simulink model "Maxom_fcs_noncascaded"  (R2025b)
settings: Solver=ode45  StartTime=0.0  StopTime=0.30  FixedStep=1e-6  MaxStep=1e-5  RelTol=1e-4  EnableMultiTasking=on
values from neighbouring files (symbols this model uses):
  Bfric = 0    [PMSMpara.m]
  ffai = 0.008667    [PMSMpara.m]
  Imax = 20    [PMSMpara.m]
  J = 0.044e-4    (= 4.4e-06)    [PMSMpara.m]
  kis = 0    [PMSMpara.m]
  kps = fsc*6.28*J/Kt    (= 0.364364007978)    [PMSMpara.m]
  Kt = np*1.5*ffai    (= 0.0910035)    [PMSMpara.m]
  Ld = Ls    (= 0.00045)    [PMSMpara.m]
  Lq = Ls    (= 0.00045)    [PMSMpara.m]
  np = 7    [PMSMpara.m]
  Rs = 0.5    [PMSMpara.m]
  Tcur = 1/32000    (= 3.125e-05)    [PMSMpara.m]
  Tpwm = 1/32000    (= 3.125e-05)    [PMSMpara.m]
  Tspd = 1/32000    (= 3.125e-05)    [PMSMpara.m]
  wn = 311040    [PMSMpara.m]
  zeta = 1    [PMSMpara.m]
undefined symbols (not defined in the file or in its folder): dspblkCoreblockFVToolHelper, gcbh
libraries: simulink x4, slpidlib x2, spsUniversalBridgeLib x1, spsCurrentMeasurementLib x1, EasyGo_Machine_lib x1, spsPermanentMagnetSynchronousMachineLib x1, spsSVPWMGenerator2LevelLib x1, spsDCVoltageSourceLib x1, sps_lib x1
(part 2 of 4)

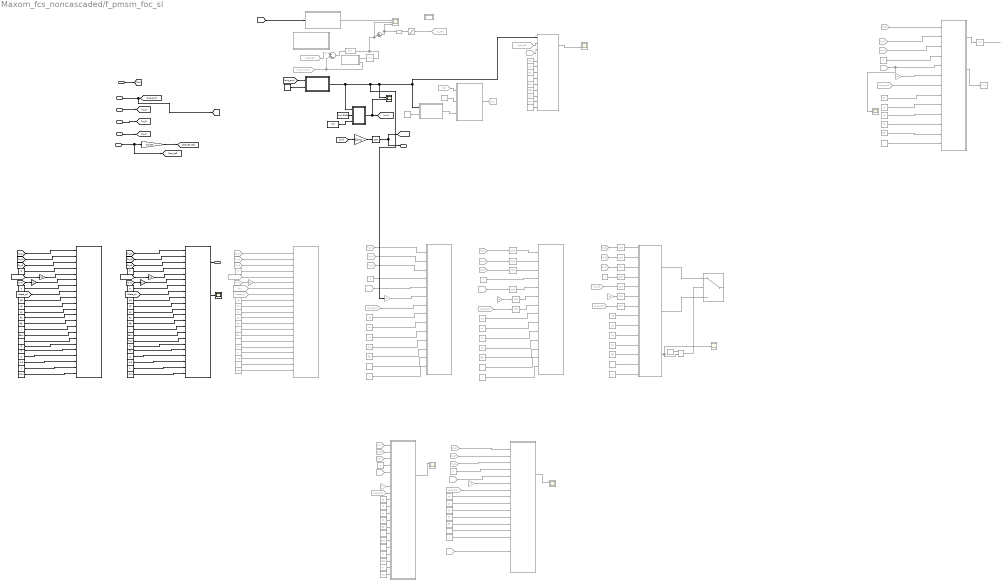
== system Maxom_fcs_noncascaded/f_pmsm_foc_sl ==
  note: This is non-cascaded, clearer to read but takes aroun 200e-6s to compute.
  note: ripple pzdc
      | but needs 20e-6 to calculate ggs
  note: 速度环控制器+电流前馈
  note: computational time around 200ms. good performance, however still the ripple ~20% exists
  note: performance same as smdo+1step, but has apendix
  note: same as the one on the right but loops were optimized and the matrix multiplication was taken out 70e-6s to compute, a little worse performn.
  Is_A : Inport  SampleTime=Tpwm
  Is_B : Inport  Port=2  SampleTime=Tpwm
  Is_C : Inport  Port=3  SampleTime=Tpwm
  ang_enc : Inport  Port=4  OutDataTypeStr=single  SampleTime=Tpwm
  spd_ref : Inport  Port=5  SampleTime=Tpwm
  Te : Inport  Port=6  SampleTime=Tpwm
  " lpf_2nd3" : Subsystem  mask{ts=Tpwm}
      mask prompts: ts "Sample time"
      mask DialogControl DescGroupVar Prompt: 2nd order low-pass filter
  Constant{,55,69,74} (4 alike) : Constant  Commented=on  Value=J
  Constant{1,5,21,24,33,45,62} (7 alike) : Constant  Commented=on  Value=Ld
  Constant{2,10,19,22,25,34,66} (7 alike) : Constant  Commented=on  Value=Lq
  Constant100 : Constant  Value=ffai
  Constant101 : Constant  Value=48
  Constant{86,90,94,102,106,110} (6 alike) : Constant  Value=0
  Constant103 : Constant  Value=Bfric
  Constant104 : Constant  Value=J
  Constant105 : Constant  Value=5
  Constant107 : Constant  Value=0.8
  Constant108 : Constant
  Constant109 : Constant  Value=Imax
  Constant{3,11,20,26,35,46,67} (7 alike) : Constant  Commented=on  Value=Rs
  Constant111 : Constant  Value=3
  Constant{4,12,27,36,40,48,58,68} (8 alike) : Constant  Commented=on  Value=Tpwm
  Constant{13,37,41,49,78} (5 alike) : Constant  Commented=on
  Constant{6,14,29,38,42,50,60,70} (8 alike) : Constant  Commented=on  Value=ffai
  Constant{7,15,30,39,43,51,71} (7 alike) : Constant  Commented=on  Value=48
  Constant{8..9,16,23,32,44,72,76} (8 alike) : Constant  Commented=on  Value=0
  Constant17 : Constant  Value=2*pi*6000  OutDataTypeStr=single
  Constant18 : Constant  Value=0.8  OutDataTypeStr=single
  Constant28 : Constant  Commented=on  Value=2
  Constant31 : Constant  Value=Tpwm  OutDataTypeStr=single
  Constant47 : Constant  Commented=on  Value=Bfric
  Constant52 : Constant  Commented=on  Value=zeta
  Constant53 : Constant  Commented=on  Value=wn
  Constant54 : Constant  Commented=on  Value=Imax
  Constant56 : Constant  Commented=on  Value=Tpwm  OutDataTypeStr=single
  Constant57 : Constant  Commented=on  Value=kis
  Constant59 : Constant  Commented=on  Value=Imax
  Constant61 : Constant  Commented=on  Value=kps
  Constant63 : Constant  Commented=on  Value=Bfric
  Constant64 : Constant  Commented=on  Value=zeta
  Constant65 : Constant  Commented=on  Value=wn
  Constant73 : Constant  Commented=on  Value=Bfric
  Constant75 : Constant  Commented=on  Value=5
  Constant77 : Constant  Commented=on  Value=0.8
  Constant79 : Constant  Commented=on  Value=Imax
  Constant80 : Constant  Value=Ld
  Constant81 : Constant  Value=Lq
  Constant82 : Constant  Value=Rs
  Constant83 : Constant  Value=Tcur
  Constant84 : Constant  Value=ffai
  Constant85 : Constant  Value=48
  Constant87 : Constant  Value=Bfric
  Constant88 : Constant  Value=J
  Constant89 : Constant  Value=5
  Constant91 : Constant  Value=0.8
  Constant92 : Constant
  Constant93 : Constant  Value=Imax
  Constant95 : Constant  Value=3
  Constant96 : Constant  Value=Ld
  Constant97 : Constant  Value=Lq
  Constant98 : Constant  Value=Rs
  Constant99 : Constant  Value=Tpwm
  Data Type Conversion : DataTypeConversion  Commented=on  SaturateOnIntegerOverflow=off  RndMeth=Floor
  Delay1 : Delay  Commented=on  DelayLength=1  InitialCondition=0  SampleTime=Tpwm
  Delay2 : Delay  Commented=on  DelayLength=1  InitialCondition=0  SampleTime=Tcur
  Delay3 : Delay  Commented=on  DelayLength=1  InitialCondition=0  SampleTime=Tcur
  Filter_13k : Subsystem  Tag=FilterWizardSubSystem  Commented=on
      settings: ErrorFcn=dspFilterRealizedInBasicElemsAlgLoopErrFcnCallback
  From{,13..14,26} (4 alike) : From  Commented=on  GotoTag=spd_ref
  From{1,6,17,21,24,31,37} (7 alike) : From  Commented=on  GotoTag=is_c
  From10 : From  Commented=on  GotoTag=wm_syn_rpm  TagVisibility=global
  From{5,12,36,42..43} (5 alike) : From  Commented=on  GotoTag=iq_ref
  From15 : From  Commented=on  GotoTag=wm
  From{2,7,18,22,28,32,38} (7 alike) : From  Commented=on  GotoTag=is_a
  From{3,8,19,23,29,33,39} (7 alike) : From  Commented=on  GotoTag=is_b
  From{4,9,20,25,35,41} (6 alike) : From  Commented=on  GotoTag=ang_enc
  From27 : From  Commented=on  GotoTag=T_load
  From30 : From  Commented=on  GotoTag=theta_e
  From34 : From  Commented=on  GotoTag=spd_ref_rad
  From40 : From  Commented=on  GotoTag=TL
  From44 : From  Commented=on  GotoTag=Te
  Gain{1..4,7,10,16} (7 alike) : Gain  Commented=on  Gain=np
  Gain14 : Gain  Gain=60/np
  Gain26 : Gain  Gain=2*pi/60
  Gain5 : Gain  Gain=np*0.895
  Gain6 : Gain  Gain=np
  Gain8 : Gain  Gain=np*0.9
  Gain9 : Gain  Gain=np
  Goto10 : Goto  Commented=on  GotoTag=iq_ref
  Goto2 : Goto  Commented=on  GotoTag=TL
  MATLAB Function : MATLAB Function  Commented=on  TreatAsAtomicUnit=on
  MATLAB Function1 : MATLAB Function  Commented=on  TreatAsAtomicUnit=on
  MATLAB Function10 : MATLAB Function  Commented=on  TreatAsAtomicUnit=on  SystemSampleTime=1/16000
  MATLAB Function11 : MATLAB Function  Commented=on  TreatAsAtomicUnit=on
  MATLAB Function12 : MATLAB Function  TreatAsAtomicUnit=on  SystemSampleTime=Tpwm
  MATLAB Function13 : MATLAB Function  TreatAsAtomicUnit=on  SystemSampleTime=Tpwm
  MATLAB Function2 : MATLAB Function  Commented=on  TreatAsAtomicUnit=on
  MATLAB Function3 : MATLAB Function  Commented=on  TreatAsAtomicUnit=on
  MATLAB Function4 : MATLAB Function  Commented=on  TreatAsAtomicUnit=on  SystemSampleTime=1/16000
  MATLAB Function5 : MATLAB Function  Commented=on  TreatAsAtomicUnit=on  SystemSampleTime=1/16000
  MATLAB Function6 : MATLAB Function  TreatAsAtomicUnit=on
  MATLAB Function7 : MATLAB Function  Commented=on  TreatAsAtomicUnit=on
  MATLAB Function8 : MATLAB Function  Commented=on  TreatAsAtomicUnit=on  SystemSampleTime=1/16000
  MATLAB Function9 : MATLAB Function  Commented=on  TreatAsAtomicUnit=on
  PID Controller : slpidlib/PID Controller  Commented=on  Controller=PI  Form=Parallel  TimeDomain=Discrete-time  UseExternalTs=off  SampleTime=Tpwm  IntegratorMethod=Forward Euler  FilterMethod=Forward Euler  ControllerParametersSource=internal  P=0.044e-4*2*pi*2500  I=0.0001*4.5*0.2*2*10  UseKiTs=off  D=0  UseExternalDerivativeSource=off  N=100  UseFilter=on  TunerSelectOption=Transfer Function Based (PID Tuner App)  InitialConditionSource=internal  InitialConditionForIntegrator=0  InitialConditionForFilter=0  DifferentiatorICPrevScaledInput=0  ExternalReset=none  TrackingMode=off  Kt=1  LimitOutput=on  SatLimitsSource=internal  UpperSaturationLimit=20  LowerSaturationLimit=-20  LinearizeAsGain=on  AntiWindupMode=clamping  Kb=0.1  LimitIntegrator=off  UpperIntegratorSaturationLimit=20  LowerIntegratorSaturationLimit=-20  POutMin=[]  POutMax=[]  IOutMin=[]  IOutMax=[]  DOutMin=[]  DOutMax=[]  NOutMin=[]  NOutMax=[]  SumOutMin=[]  SumOutMax=[]  SaturationOutMin=[]  SaturationOutMax=[]  PParamMin=[]  PParamMax=[]  IParamMin=[]  IParamMax=[]  DParamMin=[]  DParamMax=[]  NParamMin=[]  NParamMax=[]  KbParamMin=[]  KbParamMax=[]  KtParamMin=[]  KtParamMax=[]  KbOutMin=[]  KbOutMax=[]  KtOutMin=[]  KtOutMax=[]  IntegratorOutMin=[]  IntegratorOutMax=[]  FilterOutMin=[]  FilterOutMax=[]  SumI1OutMin=[]  SumI1OutMax=[]  SumI2OutMin=[]  SumI2OutMax=[]  SumI3OutMin=[]  SumI3OutMax=[]  SumI4OutMin=[]  SumI4OutMax=[]  SumDOutMin=[]  SumDOutMax=[]  DifferentiatorOutMin=[]  DifferentiatorOutMax=[]  FilterDiffOutCoefMin=[]  FilterDiffOutCoefMax=[]  ReciprocalOutMin=[]  ReciprocalOutMax=[]  SumDenOutMin=[]  SumDenOutMax=[]  SumNumOutMin=[]  SumNumOutMax=[]  DivideOutMin=[]  DivideOutMax=[]  UdiffTsProdOutMin=[]  UdiffTsProdOutMax=[]  NTsProdOutMin=[]  NTsProdOutMax=[]  UintegralTsProdOutMin=[]  UintegralTsProdOutMax=[]  UngainTsProdOutMin=[]  UngainTsProdOutMax=[]  ClampingZeroOutDataTypeStr=Inherit: Inherit via back propagation  ClampingZeroOutMin=[]  ClampingZeroOutMax=[]  FilterDenConstantOutDataTypeStr=Inherit: Inherit via back propagation  FilterDenConstantOutMin=[]  FilterDenConstantOutMax=[]  PCopyOutDataTypeStr=Inherit: Inherit via back propagation  PCopyOutMin=[]  PCopyOutMax=[]  NCopyOutDataTypeStr=Inherit: Inherit via back propagation  NCopyOutMin=[]  NCopyOutMax=[]  IntegratorContinuousStateAttributes=''  IntegratorStateMustResolveToSignalObject=off  IntegratorRTWStateStorageClass=Auto  FilterContinuousStateAttributes=''  FilterStateMustResolveToSignalObject=off  FilterRTWStateStorageClass=Auto  ParallelPVariant=InternalParameters  IdealPVariant=Disabled  IVariant=InternalParameters  DVariant=Disabled  IntegratorVariant=Discrete  SatVariant=Enabled  AWVariant=DiscClampingParallel  PCopyVariant=Disabled  TRVariant=Disabled  FdbkBlocksVariant=Forward  IdealPFdbkVariant=Disabled  SatFdbkVariant=Disabled  DerivativeFilterVariant=Disabled  NVariant=Disabled  NCopyVariant=Disabled_SignalSpec  FilterICVariant=Disabled  IntegratorICVariant=InternalICs  ExternalResetVariant=Disabled  TRSumVariant=Passthrough  SumFdbkVariant=Disabled  SumVariant=Sum_PI  TsampFilterVariant=InternalTs  TsampNgainVariant=Passthrough  TsampIntegralVariant=Disabled_SignalSpec  ExternalSaturationOutDataTypeStr=Inherit: Same as second input  DerivativeSourceVariant=Disabled  PreIntVariant=InternalPreInt
  Relational Operator : RelationalOperator  Commented=on  Operator=<  OutDataTypeStr=boolean  RndMeth=Simplest  InputSameDT=off
  Repeating Sequence2 : simulink/Sources/Repeating Sequence  Commented=on  rep_seq_t=[0 Tpwm]  rep_seq_y=[0 1]
  Saturation : Saturate  Commented=on  UpperLimit=20  LowerLimit=-20
  Scope : Scope  Commented=on  NumInputPorts=3
      settings: ActiveDisplayYMinimum=-24.249076789999609  ActiveDisplayYMaximum=20.144440314798036
  Scope1 : Scope  Commented=on
      settings: ActiveDisplayYMinimum=-1  ActiveDisplayYMaximum=1
  Scope10 : Scope  Commented=on
      settings: ActiveDisplayYMinimum=-0.40417617181618054  ActiveDisplayYMaximum=1.3464253644677231  DataLoggingVariableName=ScopeData2
  Scope2 : Scope  Commented=on  NumInputPorts=2
      settings: ActiveDisplayYMinimum=-28.042138576507568  ActiveDisplayYMaximum=28.086816310882568  DataLoggingVariableName=ScopeData6
  Scope3 : Scope  Commented=on  NumInputPorts=2
      settings: ActiveDisplayYMinimum=-28.042138576507568  ActiveDisplayYMaximum=28.086816310882568  DataLoggingVariableName=ScopeData7
  Scope4 : Scope  Commented=on  NumInputPorts=2
      settings: ActiveDisplayYMinimum=-27.5888969521045  ActiveDisplayYMaximum=22.4111030478955
  Scope5 : Scope  NumInputPorts=2
      settings: ActiveDisplayYMinimum=-369.62545776367188  ActiveDisplayYMaximum=368.15011596679688  DataLoggingVariableName=ScopeData2
  Scope6 : Scope
      settings: ActiveDisplayYMinimum=-59.477871894836426  ActiveDisplayYMaximum=60.065136909484863  DataLoggingVariableName=ScopeData8
  Subsystem3 : Subsystem  Commented=on
  Sum : Sum  Commented=on  Inputs=|+--
  Sum6 : Sum  Commented=on  Inputs=|+++
  Switch : Switch  Commented=on  Criteria=u2 > Threshold  SaturateOnIntegerOverflow=off  InputSameDT=off
  Zero-Order Hold10 : ZeroOrderHold  SampleTime=Tpwm
  Zero-Order Hold{19..31} (13 alike) : ZeroOrderHold  Commented=on  SampleTime=Tpwm
  original1 : MATLAB Function  Commented=on  TreatAsAtomicUnit=on
  Out2 : Outport
  gg : Outport  Port=2
  tag scope: wm_syn_rpm=global
  wires:
  Is_A/1 -> [is_a]
  Is_B/1 -> [is_b]
  Is_C/1 -> [is_c]
  spd_ref/1 -> [spd_ref], Gain26/1
  Sum/1 -> PID Controller/1
  From13/1 -> Sum/1
  Delay1/1 -> Subsystem3/1(iq)
  From10/1 -> Subsystem3/2(spd), Sum/2
  Gain26/1 -> [spd_ref_rad]
  PID Controller/1 -> Scope/2, Sum6/2, Delay1/1
  Constant18/1 -> " lpf_2nd3"/3(zeta)
  Constant17/1 -> " lpf_2nd3"/2(wn)
  " lpf_2nd3"/1(y) -> Scope5/2, [wm]
  MATLAB Function1/1(iq_feedforward) -> Scope/1
  Sum6/1 -> Data Type Conversion/1, Scope/3
  Data Type Conversion/1 -> Saturation/1
  Saturation/1 -> Goto10/1
  [ang_enc] -> MATLAB Function6/1(theta_e)
  Constant31/1 -> MATLAB Function6/2(Ts)
  [wm] -> Gain14/1
  Gain14/1 -> Zero-Order Hold10/1
  Zero-Order Hold10/1 -> Out2/1, [wm_syn_rpm]
  Zero-Order Hold19/1 -> MATLAB Function7/1(ia)
  Zero-Order Hold23/1 -> MATLAB Function7/7(theta_mech)
  Constant36/1 -> MATLAB Function7/13(Tcur)
  Zero-Order Hold20/1 -> MATLAB Function7/2(ib)
  From31/1 -> Zero-Order Hold24/1
  Constant37/1 -> MATLAB Function7/14(lambda_w)
  Gain16/1 -> Zero-Order Hold22/1
  Constant35/1 -> MATLAB Function7/11(Rs)
  From32/1 -> Zero-Order Hold19/1
  Zero-Order Hold22/1 -> MATLAB Function7/6(omega_mech)
  From35/1 -> Zero-Order Hold23/1
  Zero-Order Hold21/1 -> MATLAB Function7/5(iq_ref)
  From36/1 -> Zero-Order Hold21/1
  Constant33/1 -> MATLAB Function7/9(Ld)
  Constant34/1 -> MATLAB Function7/10(Lq)
  Constant39/1 -> MATLAB Function7/8(Vdc)
  Constant32/1 -> MATLAB Function7/4(id_ref)
  Zero-Order Hold24/1 -> MATLAB Function7/3(ic)
  From33/1 -> Zero-Order Hold20/1
  Constant38/1 -> MATLAB Function7/12(lambda_f)
  From39/1 -> MATLAB Function5/2(ib)
  Constant9/1 -> MATLAB Function5/4(id_ref)
  Constant46/1 -> MATLAB Function5/11(Rs)
  From42/1 -> MATLAB Function5/5(iq_ref)
  Gain10/1 -> MATLAB Function5/6(omega_mech)
  From41/1 -> MATLAB Function5/7(theta_mech)
  From38/1 -> MATLAB Function5/1(ia)
  Constant49/1 -> MATLAB Function5/14(lambda_w)
  Constant22/1 -> MATLAB Function5/10(Lq)
  Constant21/1 -> MATLAB Function5/9(Ld)
  Constant51/1 -> MATLAB Function5/8(Vdc)
  Constant50/1 -> MATLAB Function5/12(lambda_f)
  Constant48/1 -> MATLAB Function5/13(Tcur)
  From37/1 -> MATLAB Function5/3(ic)
  Repeating Sequence2/1 -> Relational Operator/1
  original1/2(gB) -> Switch/3
  From22/1 -> Zero-Order Hold25/1
  Constant25/1 -> original1/10(Lq)
  Constant29/1 -> original1/12(lambda_f)
  Constant24/1 -> original1/9(Ld)
  Constant28/1 -> original1/14(lambda_w)
  Zero-Order Hold30/1 -> original1/3(ic)
  Constant26/1 -> original1/11(Rs)
  Relational Operator/1 -> Switch/2
  Gain7/1 -> Zero-Order Hold28/1
  Zero-Order Hold27/1 -> original1/4(id_ref)
  Zero-Order Hold26/1 -> original1/2(ib)
  Zero-Order Hold28/1 -> original1/6(omega_mech)
  From25/1 -> Zero-Order Hold29/1
  original1/1(gA) -> Switch/1
  From21/1 -> Zero-Order Hold30/1
  Constant30/1 -> original1/8(Vdc)
  Zero-Order Hold31/1 -> original1/5(iq_ref)
  Constant23/1 -> Zero-Order Hold27/1
  Zero-Order Hold25/1 -> original1/1(ia)
  From23/1 -> Zero-Order Hold26/1
  Constant27/1 -> original1/13(Tpwm)
  original1/3(d) -> Relational Operator/2, Scope10/1
  From43/1 -> Zero-Order Hold31/1
  Zero-Order Hold29/1 -> original1/7(theta_mech)
  Constant4/1 -> MATLAB Function2/13(Tcur)
  From2/1 -> MATLAB Function2/1(ia)
  Constant2/1 -> MATLAB Function2/10(Lq)
  From1/1 -> MATLAB Function2/3(ic)
  From5/1 -> Scope1/1, MATLAB Function2/5(iq_ref)
  Constant6/1 -> MATLAB Function2/12(lambda_f)
  From3/1 -> MATLAB Function2/2(ib)
  Constant7/1 -> MATLAB Function2/8(Vdc)
  Constant1/1 -> MATLAB Function2/9(Ld)
  Constant3/1 -> MATLAB Function2/11(Rs)
  Constant8/1 -> MATLAB Function2/4(id_ref)
  Gain1/1 -> MATLAB Function2/6(omega_mech)
  From4/1 -> MATLAB Function2/7(theta_mech)
  MATLAB Function2/1(v_alpha) -> Delay3/1
  MATLAB Function2/2(v_beta) -> Delay2/1
  Delay3/1 -> ?
  Constant12/1 -> MATLAB Function4/13(Tcur)
  Constant15/1 -> MATLAB Function4/8(Vdc)
  From8/1 -> MATLAB Function4/2(ib)
  Constant16/1 -> MATLAB Function4/4(id_ref)
  Constant10/1 -> MATLAB Function4/10(Lq)
  From7/1 -> MATLAB Function4/1(ia)
  From6/1 -> MATLAB Function4/3(ic)
  Constant11/1 -> MATLAB Function4/11(Rs)
  Constant5/1 -> MATLAB Function4/9(Ld)
  From12/1 -> MATLAB Function4/5(we_ref)
  Constant14/1 -> MATLAB Function4/12(lambda_f)
  Gain2/1 -> MATLAB Function4/6(we)
  From9/1 -> MATLAB Function4/7(theta_mech)
  From/1 -> MATLAB Function4/16(Ki_we)
  Constant13/1 -> MATLAB Function4/14(lambda_c)
  MATLAB Function4/1(i_pred) -> Scope2/1
  MATLAB Function8/1(i_pred) -> Scope3/1
  Constant42/1 -> MATLAB Function8/13(lambda_f)
  Constant40/1 -> MATLAB Function8/16(Tcur)
  Constant41/1 -> MATLAB Function8/17(lambda_c)
  Constant20/1 -> MATLAB Function8/12(Rs)
  Constant19/1 -> MATLAB Function8/11(Lq)
  Constant45/1 -> MATLAB Function8/10(Ld)
  Constant43/1 -> MATLAB Function8/9(Vdc)
  From20/1 -> MATLAB Function8/8(theta_mech)
  Gain3/1 -> MATLAB Function8/7(we)
  From14/1 -> MATLAB Function8/5(we_ref)
  Constant44/1 -> MATLAB Function8/4(id_ref)
  From17/1 -> MATLAB Function8/3(ic)
  From18/1 -> MATLAB Function8/1(ia)
  From19/1 -> MATLAB Function8/2(ib)
  Constant/1 -> MATLAB Function8/14(Jm)
  Constant47/1 -> MATLAB Function8/15(Bfric)
  Constant52/1 -> MATLAB Function8/18(zeta)
  Constant53/1 -> MATLAB Function8/19(wn)
  Constant54/1 -> MATLAB Function8/20(iq_max)
  Te/1 -> [Te]
  ? -> MATLAB Function8/6(TL_hat)
  Constant58/1 -> MATLAB Function/13(Tcur)
  Constant64/1 -> MATLAB Function/10(zeta)
  Constant55/1 -> MATLAB Function/8(Jm)
  Constant60/1 -> MATLAB Function/7(lambda_f)
  From26/1 -> MATLAB Function/2(we_ref)
  Constant65/1 -> MATLAB Function/11(wn)
  Constant59/1 -> MATLAB Function/12(iq_max)
  Constant63/1 -> MATLAB Function/9(Bfric)
  From27/1 -> MATLAB Function/3(Te)
  MATLAB Function/1(iq_ref) -> Scope4/2
  Constant56/1 -> MATLAB Function9/2(Ts)
  Constant57/1 -> MATLAB Function/6(Kis)
  Constant61/1 -> MATLAB Function/5(Kps)
  Constant62/1 -> MATLAB Function10/10(Ld)
  Constant68/1 -> MATLAB Function10/16(Tcur)
  Constant71/1 -> MATLAB Function10/9(Vdc)
  From29/1 -> MATLAB Function10/2(ib)
  Constant72/1 -> MATLAB Function10/4(id_ref)
  Constant66/1 -> MATLAB Function10/11(Lq)
  From28/1 -> MATLAB Function10/1(ia)
  From24/1 -> MATLAB Function10/3(ic)
  Constant67/1 -> MATLAB Function10/12(Rs)
  From34/1 -> MATLAB Function10/5(we_ref)
  Constant70/1 -> MATLAB Function10/13(lambda_f)
  Gain4/1 -> MATLAB Function10/6(we)
  From30/1 -> MATLAB Function10/8(theta_m)
  From40/1 -> MATLAB Function10/7(TL_hat)
  MATLAB Function6/1(we_raw) -> " lpf_2nd3"/1(u), Gain10/1, Scope5/1, MATLAB Function9/1(we), MATLAB Function/1(we)
  Constant73/1 -> MATLAB Function10/15(Bfric)
  Constant74/1 -> MATLAB Function10/14(Jm)
  Constant75/1 -> MATLAB Function10/17(lambda_id)
  Constant76/1 -> MATLAB Function10/18(lambda_sw)
  Constant77/1 -> MATLAB Function10/19(we_scale)
  Constant78/1 -> MATLAB Function10/20(i_scale)
  Constant79/1 -> MATLAB Function10/21(iq_max)
  From44/1 -> MATLAB Function11/1(Te)
  Constant69/1 -> MATLAB Function11/2(J)
  MATLAB Function9/1(we_dot) -> MATLAB Function11/3(wm_hat)
  MATLAB Function11/1(TL) -> Goto2/1
  ang_enc/1 -> [theta_e], [ang_enc]
  From15/1 -> Gain4/1
  [wm] -> Gain5/1
  Constant85/1 -> MATLAB Function12/9(Vdc)
  Constant80/1 -> MATLAB Function12/10(Ld)
  Constant83/1 -> MATLAB Function12/16(Tcur)
  Constant91/1 -> MATLAB Function12/20(we_scale)
  Constant87/1 -> MATLAB Function12/15(Bfric)
  Constant89/1 -> MATLAB Function12/18(lambda_id)
  Constant82/1 -> MATLAB Function12/12(Rs)
  Constant92/1 -> MATLAB Function12/21(i_scale)
  [spd_ref_rad] -> Gain6/1
  Constant94/1 -> MATLAB Function12/7(TL_hat)
  [is_b] -> MATLAB Function12/2(ib)
  [theta_e] -> MATLAB Function12/8(theta_m)
  Gain5/1 -> MATLAB Function12/6(we)
  Constant84/1 -> MATLAB Function12/13(lambda_f)
  Constant93/1 -> MATLAB Function12/22(iq_max)
  Constant86/1 -> MATLAB Function12/4(id_ref)
  Constant88/1 -> MATLAB Function12/14(Jm)
  [is_a] -> MATLAB Function12/1(ia)
  [is_c] -> MATLAB Function12/3(ic)
  Constant81/1 -> MATLAB Function12/11(Lq)
  Constant90/1 -> MATLAB Function12/19(lambda_sw)
  Gain6/1 -> MATLAB Function12/5(we_ref)
  Constant95/1 -> MATLAB Function12/17(lambda_w)
  [is_b] -> MATLAB Function13/2(ib)
  Constant102/1 -> MATLAB Function13/4(id_ref)
  Gain8/1 -> MATLAB Function13/6(we)
  Constant111/1 -> MATLAB Function13/17(lambda_w)
  [is_a] -> MATLAB Function13/1(ia)
  Constant98/1 -> MATLAB Function13/12(Rs)
  Constant97/1 -> MATLAB Function13/11(Lq)
  Constant107/1 -> MATLAB Function13/20(we_scale)
  [wm] -> Gain8/1
  Constant104/1 -> MATLAB Function13/14(Jm)
  Constant108/1 -> MATLAB Function13/21(i_scale)
  Constant99/1 -> MATLAB Function13/16(Tcur)
  Constant103/1 -> MATLAB Function13/15(Bfric)
  Constant110/1 -> MATLAB Function13/7(TL_hat)
  Constant101/1 -> MATLAB Function13/9(Vdc)
  Constant96/1 -> MATLAB Function13/10(Ld)
  Constant105/1 -> MATLAB Function13/18(lambda_id)
  Gain9/1 -> MATLAB Function13/5(we_ref)
  [theta_e] -> MATLAB Function13/8(theta_m)
  [spd_ref_rad] -> Gain9/1
  [is_c] -> MATLAB Function13/3(ic)
  Constant109/1 -> MATLAB Function13/22(iq_max)
  Constant106/1 -> MATLAB Function13/19(lambda_sw)
  Constant100/1 -> MATLAB Function13/13(lambda_f)
  [spd_ref] -> MATLAB Function1/1(speed_ref_cmd)
  MATLAB Function12/1(gg) -> gg/1
  MATLAB Function12/2(i_pred) -> Scope6/1

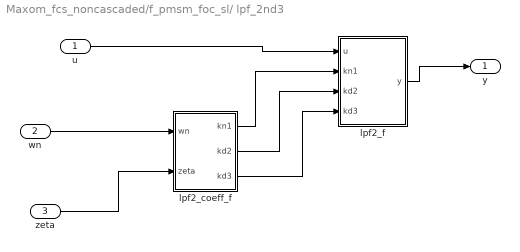
== system Maxom_fcs_noncascaded/f_pmsm_foc_sl/ lpf_2nd3 ==
  u : Inport  SampleTime=ts
  wn : Inport  Port=2  SampleTime=ts
  zeta : Inport  Port=3  SampleTime=ts
  lpf2_coeff_f : Subsystem
  lpf2_f : Subsystem
  y : Outport
  wires:
  wn/1 -> lpf2_coeff_f/1(wn)
  lpf2_f/1(y) -> y/1
  lpf2_coeff_f/3(kd3) -> lpf2_f/4(kd3)
  zeta/1 -> lpf2_coeff_f/2(zeta)
  lpf2_coeff_f/1(kn1) -> lpf2_f/2(kn1)
  lpf2_coeff_f/2(kd2) -> lpf2_f/3(kd2)
  u/1 -> lpf2_f/1(u)

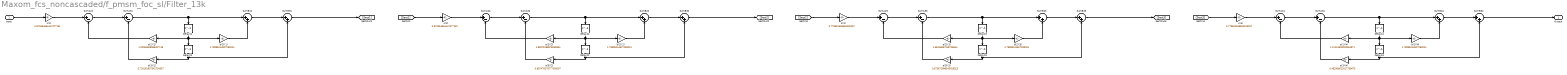
== system Maxom_fcs_noncascaded/f_pmsm_foc_sl/Filter_13k ==
  Input : Inport
  Delay{11..14,21..24} (8 alike) : Delay  DelayLength=1  InitialCondition=0
  SumA{21..24,31..34} (8 alike) : Sum  Inputs=|+-  RndMeth=Nearest  SaturateOnIntegerOverflow=on  OutDataTypeStr=Inherit: Same as first input
  SumB{21..24,31..34} (8 alike) : Sum  Inputs=|++  RndMeth=Nearest  SaturateOnIntegerOverflow=on  OutDataTypeStr=Inherit: Same as first input
  a(2)(1) : Gain  Gain=1.20064608086497748  ParamDataTypeStr=double  RndMeth=Nearest  SaturateOnIntegerOverflow=on  OutDataTypeStr=Inherit: Same as input
  a(2)(2) : Gain  Gain=1.83979198876035954  ParamDataTypeStr=double  RndMeth=Nearest  SaturateOnIntegerOverflow=on  OutDataTypeStr=Inherit: Same as input
  a(2)(3) : Gain  Gain=1.58416837048726844  ParamDataTypeStr=double  RndMeth=Nearest  SaturateOnIntegerOverflow=on  OutDataTypeStr=Inherit: Same as input
  a(2)(4) : Gain  Gain=1.21113909228264971  ParamDataTypeStr=double  RndMeth=Nearest  SaturateOnIntegerOverflow=on  OutDataTypeStr=Inherit: Same as input
  a(3)(1) : Gain  Gain=0.726162637542734357  ParamDataTypeStr=double  RndMeth=Nearest  SaturateOnIntegerOverflow=on  OutDataTypeStr=Inherit: Same as input
  a(3)(2) : Gain  Gain=0.897478278777509297  ParamDataTypeStr=double  RndMeth=Nearest  SaturateOnIntegerOverflow=on  OutDataTypeStr=Inherit: Same as input
  a(3)(3) : Gain  Gain=0.673672996545029323  ParamDataTypeStr=double  RndMeth=Nearest  SaturateOnIntegerOverflow=on  OutDataTypeStr=Inherit: Same as input
  a(3)(4) : Gain  Gain=0.482908022017759675  ParamDataTypeStr=double  RndMeth=Nearest  SaturateOnIntegerOverflow=on  OutDataTypeStr=Inherit: Same as input
  b(2)(1) : Gain  Gain=1.79995244627283024  ParamDataTypeStr=double  RndMeth=Nearest  SaturateOnIntegerOverflow=on  OutDataTypeStr=Inherit: Same as input
  b(2)(2) : Gain  Gain=1.79995244627283024  ParamDataTypeStr=double  RndMeth=Nearest  SaturateOnIntegerOverflow=on  OutDataTypeStr=Inherit: Same as input
  b(2)(3) : Gain  Gain=1.79995244627283024  ParamDataTypeStr=double  RndMeth=Nearest  SaturateOnIntegerOverflow=on  OutDataTypeStr=Inherit: Same as input
  b(2)(4) : Gain  Gain=1.79995244627283024  ParamDataTypeStr=double  RndMeth=Nearest  SaturateOnIntegerOverflow=on  OutDataTypeStr=Inherit: Same as input
  s(1) : Gain  Gain=0.870354664447377191  ParamDataTypeStr=double  RndMeth=Nearest  SaturateOnIntegerOverflow=on  OutDataTypeStr=Inherit: Same as input
  s(2) : Gain  Gain=0.870354664447377191  ParamDataTypeStr=double  RndMeth=Nearest  SaturateOnIntegerOverflow=on  OutDataTypeStr=Inherit: Same as input
  s(3) : Gain  Gain=0.779631536553225257  ParamDataTypeStr=double  RndMeth=Nearest  SaturateOnIntegerOverflow=on  OutDataTypeStr=Inherit: Same as input
  s(4) : Gain  Gain=0.779631536553225257  ParamDataTypeStr=double  RndMeth=Nearest  SaturateOnIntegerOverflow=on  OutDataTypeStr=Inherit: Same as input
  Output : Outport
  wires:
  Input/1 -> s(1)/1
  s(1)/1 -> SumA21/1
  SumA21/1 -> SumA31/1
  SumA31/1 -> SumB21/1, Delay11/1
  SumB21/1 -> SumB31/1
  SumB31/1 -> [Sect1]
  a(2)(1)/1 -> SumA21/2
  Delay11/1 -> a(2)(1)/1, b(2)(1)/1, Delay21/1
  b(2)(1)/1 -> SumB21/2
  a(3)(1)/1 -> SumA31/2
  Delay21/1 -> a(3)(1)/1, SumB31/2
  [Sect1] -> s(2)/1
  s(2)/1 -> SumA22/1
  SumA22/1 -> SumA32/1
  SumA32/1 -> SumB22/1, Delay12/1
  SumB22/1 -> SumB32/1
  SumB32/1 -> [Sect2]
  a(2)(2)/1 -> SumA22/2
  Delay12/1 -> a(2)(2)/1, b(2)(2)/1, Delay22/1
  b(2)(2)/1 -> SumB22/2
  a(3)(2)/1 -> SumA32/2
  Delay22/1 -> a(3)(2)/1, SumB32/2
  [Sect2] -> s(3)/1
  s(3)/1 -> SumA23/1
  SumA23/1 -> SumA33/1
  SumA33/1 -> SumB23/1, Delay13/1
  SumB23/1 -> SumB33/1
  SumB33/1 -> [Sect3]
  a(2)(3)/1 -> SumA23/2
  Delay13/1 -> a(2)(3)/1, b(2)(3)/1, Delay23/1
  b(2)(3)/1 -> SumB23/2
  a(3)(3)/1 -> SumA33/2
  Delay23/1 -> a(3)(3)/1, SumB33/2
  [Sect3] -> s(4)/1
  s(4)/1 -> SumA24/1
  SumA24/1 -> SumA34/1
  SumA34/1 -> SumB24/1, Delay14/1
  SumB24/1 -> SumB34/1
  SumB34/1 -> Output/1
  a(2)(4)/1 -> SumA24/2
  Delay14/1 -> a(2)(4)/1, b(2)(4)/1, Delay24/1
  b(2)(4)/1 -> SumB24/2
  a(3)(4)/1 -> SumA34/2
  Delay24/1 -> a(3)(4)/1, SumB34/2

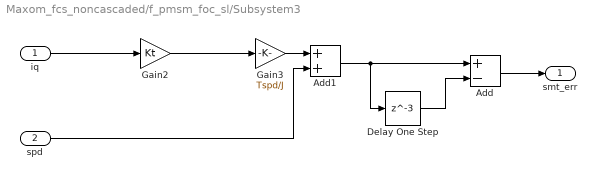
== system Maxom_fcs_noncascaded/f_pmsm_foc_sl/Subsystem3 ==
  iq : Inport
  spd : Inport  Port=2
  Add : Sum  Inputs=+-
  Add1 : Sum
  Delay One Step : Delay  DelayLength=3  SampleTime=Tpwm
  Gain2 : Gain  Gain=Kt
  Gain3 : Gain  Gain=Tspd/J
  smt_err : Outport
  wires:
  iq/1 -> Gain2/1
  spd/1 -> Add1/2
  Add1/1 -> Delay One Step/1, Add/1
  Delay One Step/1 -> Add/2
  Add/1 -> smt_err/1
  Gain2/1 -> Gain3/1
  Gain3/1 -> Add1/1

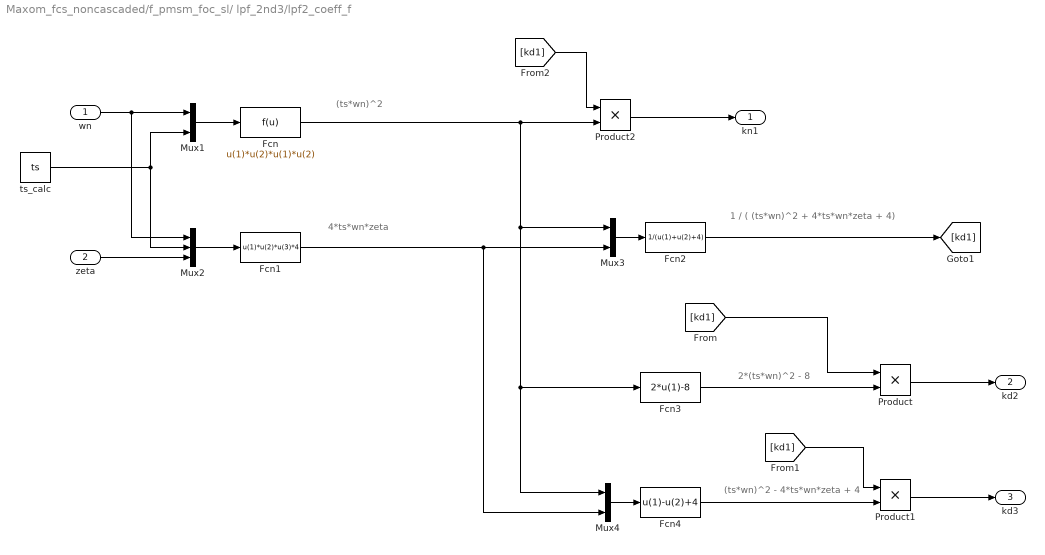
== system Maxom_fcs_noncascaded/f_pmsm_foc_sl/ lpf_2nd3/lpf2_coeff_f ==
  note: (ts*wn)^2 - 4*ts*wn*zeta + 4
  note: 4*ts*wn*zeta
  note: 2*(ts*wn)^2 - 8
  note: 1 / ( (ts*wn)^2 + 4*ts*wn*zeta + 4)
  note: (ts*wn)^2
  wn : Inport  OutDataTypeStr=single
  zeta : Inport  Port=2  OutDataTypeStr=single
  Fcn : Fcn  Expr=u(1)*u(2)*u(1)*u(2)
  Fcn1 : Fcn  Expr=u(1)*u(2)*u(3)*4
  Fcn2 : Fcn  Expr=1/(u(1)+u(2)+4)
  Fcn3 : Fcn  Expr=2*u(1)-8
  Fcn4 : Fcn  Expr=u(1)-u(2)+4
  Mux1 : Mux  Inputs=2
  Mux2 : Mux  Inputs=3
  Mux3 : Mux  Inputs=2
  Mux4 : Mux  Inputs=2
  Product : Product
  Product1 : Product
  Product2 : Product
  ts_calc : Constant  Value=ts  OutDataTypeStr=single  SampleTime=ts
  kn1 : Outport
  kd2 : Outport  Port=2
  kd3 : Outport  Port=3
  wires:
  zeta/1 -> Mux2/3
  Fcn2/1 -> [kd1]
  wn/1 -> Mux2/1, Mux1/1
  Mux1/1 -> Fcn/1
  Fcn/1 -> Product2/2, Mux4/1, Fcn3/1, Mux3/1
  Mux4/1 -> Fcn4/1
  Fcn1/1 -> Mux4/2, Mux3/2
  ts_calc/1 -> Mux2/2, Mux1/2
  Mux2/1 -> Fcn1/1
  Mux3/1 -> Fcn2/1
  [kd1] -> Product1/1
  Product/1 -> kd2/1
  [kd1] -> Product/1
  Fcn3/1 -> Product/2
  Product2/1 -> kn1/1
  Fcn4/1 -> Product1/2
  [kd1] -> Product2/1
  Product1/1 -> kd3/1

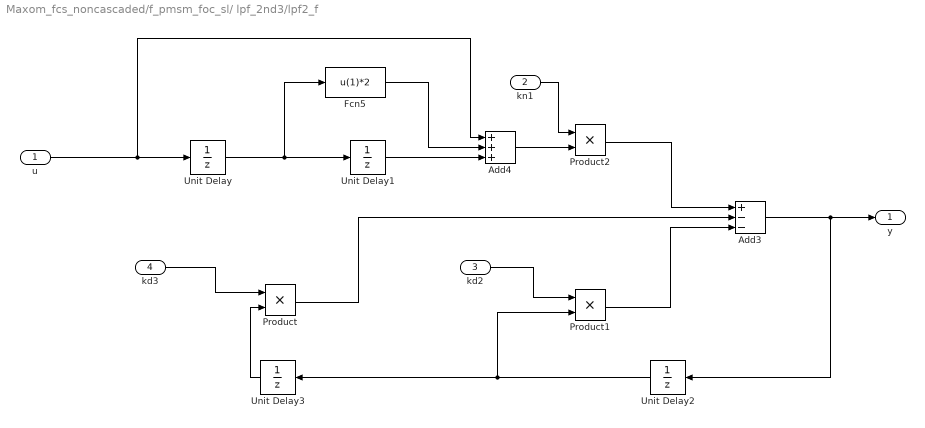
== system Maxom_fcs_noncascaded/f_pmsm_foc_sl/ lpf_2nd3/lpf2_f ==
  u : Inport  OutDataTypeStr=single  SampleTime=ts
  kn1 : Inport  Port=2  OutDataTypeStr=single
  kd2 : Inport  Port=3  OutDataTypeStr=single
  kd3 : Inport  Port=4  OutDataTypeStr=single
  Add3 : Sum  Inputs=+--
  Add4 : Sum  Inputs=+++
  Fcn5 : Fcn  Expr=u(1)*2
  Product : Product
  Product1 : Product
  Product2 : Product
  Unit Delay{,1..3} (4 alike) : UnitDelay  SampleTime=ts  HasFrameUpgradeWarning=on
  y : Outport
  wires:
  u/1 -> Unit Delay/1, Add4/1
  Unit Delay3/1 -> Product/2
  Unit Delay2/1 -> Product1/2, Unit Delay3/1
  Add4/1 -> Product2/2
  Product1/1 -> Add3/3
  Product/1 -> Add3/2
  Unit Delay/1 -> Unit Delay1/1, Fcn5/1
  kn1/1 -> Product2/1
  Unit Delay1/1 -> Add4/3
  Product2/1 -> Add3/1
  Fcn5/1 -> Add4/2
  Add3/1 -> Unit Delay2/1, y/1
  kd2/1 -> Product1/1
  kd3/1 -> Product/1

== matlab function Maxom_fcs_noncascaded/f_pmsm_foc_sl/MATLAB Function3 ==
  data: spd_ref input; iq_total output; spd_act input; iq_ff input
function iq_total = fcn_PI_FF_AntiWindup(spd_ref, spd_act, iq_ff)
    % ------------ 系统硬参数定义 ------------
    FS = single(32000);
    DT = single(1)/FS;  % 采样周期 31.25us
    Kp = single(1.5);   % 比例系数（请根据您原来 PID 的参数修改）
    Ki = single(50.0);  % 积分系数（请根据您原来 PID 的参数修改）
    
    MAX_LIM = single(20);    % 上限幅 (跟您外部的 20A 保持一致)
    MIN_LIM = single(-20);   % 下限幅
    
    persistent integral
    if isempty(integral)
        integral = single(0);
    end
    
    % 1. 计算速度误差
    error = spd_ref - spd_act;
    
    % 2. 计算 PI 输出 + 前馈 的总和
    iq_total_raw = (Kp * error + integral) + iq_ff;
    
    % 3. 对总和进行外部限幅
    if iq_total_raw > MAX_LIM
        iq_total = MAX_LIM;
    elseif iq_total_raw < MIN_LIM
        iq_total = MIN_LIM;
    else
        iq_total = iq_total_raw;
    end
    
    % 4. 【核心】：感知外部限幅的真实抗饱和策略
    % 如果触发了限幅，且误差方向还试图让限幅更深，则冻结积分器！
    if (iq_total >= MAX_LIM && error > 0) || (iq_total <= MIN_LIM && error < 0)
        integral = integral; % 冻结积分
    else
        integral = integral + Ki * error * DT; % 正常累加积分
    end
end

== matlab function Maxom_fcs_noncascaded/f_pmsm_foc_sl/MATLAB Function8 ==
  data: ia input; ib input; ic input; id_ref input; we_ref input; TL_hat input; we input; theta_mech input; Vdc input; Ld input; Lq input; Rs input; lambda_f input; Jm input; Bfric input; Tcur input; lambda_c input; i_pred output; gg output; zeta input; wn input; iq_max input
function [i_pred, gg] = fcs_smdo_1s_we_with_torque( ...
    ia, ib, ic, id_ref, we_ref, TL_hat, we, theta_mech, ...
    Vdc, Ld, Lq, Rs, lambda_f, Jm, Bfric, ...
    Tcur, lambda_c, zeta, wn, iq_max)
%#codegen
%
% we, we_ref : electrical angular speed [rad/s]
% theta_mech : mechanical rotor angle [rad]
% TL_hat     : estimated load torque [N*m]
% wn         : speed-loop natural frequency [rad/s]
% zeta       : damping ratio, normally 1
% Jm         : mechanical inertia [kg*m^2]
% Bfric      : viscous-friction coefficient
% np         : number of pole pairs
%
% Output:
% i_pred = [predicted id, predicted iq]
% gg     = six gate signals

%% Convert inputs to single precision

ia         = single(ia);
ib         = single(ib);
ic         = single(ic);

id_ref     = single(id_ref);
we_ref     = single(we_ref);
TL_hat     = single(TL_hat);
we         = single(we);
theta_mech = single(theta_mech);

Vdc        = single(Vdc);
Ld         = single(Ld);
Lq         = single(Lq);
Rs         = single(Rs);
lambda_f   = single(lambda_f);

np         = single(7);
Jm         = single(Jm);
Bfric      = single(Bfric);

Ts         = single(Tcur);
lambda_c   = single(lambda_c);

zeta       = single(zeta);
wn         = single(wn);
iq_max     = single(iq_max);

AB         = single(0.6);
BB         = single(1.2);
K1         = single(6000);
K2         = single(6000);
K3         = single(2.5e5);
K4         = single(2.5e5);

% Electrical angle

theta_e = single(mod(np*theta_mech - pi/2, 2*pi));

% Calculate torque constant and speed PI gains
Kt = 1.5*np*lambda_f;
denominator = np*Kt;
Kp_we = (single(2)*zeta*wn*Jm-Bfric)/denominator;
Ki_we = (Jm*wn*wn)/denominator;
Kaw = Ki_we / Kp_we;


% Precompute motor-model constants

inv_Ld = single(1)/Ld;
inv_Lq = single(1)/Lq;
inv_Kt = single(1)/Kt;

TsLd = Ts*inv_Ld;
TsLq = Ts*inv_Lq;

ct = single(cos(theta_e));
st = single(sin(theta_e));

sqrt3 = single(sqrt(3));

% Clarke and Park transformations

i_alpha = single(2/3)*(ia - single(0.5)*ib - single(0.5)*ic);

i_beta = single(2/3)*(sqrt3/single(2))*(ib-ic);

is_d = single( ct*i_alpha + st*i_beta);
is_q = single(-st*i_alpha + ct*i_beta);

x_k = single([is_d; is_q]);

% Inverter switching vectors

V = single([ ...
    0 0 0;
    1 0 0;
    1 1 0;
    0 1 0;
    0 1 1;
    0 0 1;
    1 0 1;
    1 1 1]);

Kcl = single(2/3)*Vdc*single([1, -0.5, -0.5; 0, sqrt3/2, -sqrt3/2]);

% Persistent controller and observer states

persistent z1 z2 s_prev Ispd

if isempty(z1)
    z1     = x_k;
    z2     = zeros(2,1,'single');
    s_prev = zeros(3,1,'single');
    Ispd   = single(0);
end

% Electrical-speed PI controller

e_we = we_ref-we;

% Load-torque feed-forward
iq_ff = TL_hat*inv_Kt;

% Complete unsaturated current command
iq_unsat = Kp_we*e_we + Ispd + iq_ff;

% Current saturation
iq_ref = max(min(iq_unsat,iq_max),-iq_max);

% Back-calculation anti-windup
Ispd = Ispd + Ts*(Ki_we*e_we + Kaw*(iq_ref-iq_unsat));

% Previous electrical angle
th_previous = theta_e-we*Ts;

ctp = single(cos(th_previous));
stp = single(sin(th_previous));
% Previously applied voltage in dq coordinates
v_app = single([ctp, stp; -stp, ctp])*(Kcl*s_prev);

% Observer error
e = z1-x_k;

ae = abs(e);
se = sign(e);

sa1 = ae.^AB .* se;
sb1 = ae.^BB .* se;

sa2 = ae.^(single(2)*AB-single(1)) .* se;
sb2 = ae.^(single(2)*BB-single(1)) .* se;

% Nominal PMSM current dynamics
f_nom = single([ (-Rs*x_k(1) + we*Lq*x_k(2))*inv_Ld;
    (-Rs*x_k(2) - we*Ld*x_k(1) - we*lambda_f)*inv_Lq]);

% Applied voltage term
g_u = single([v_app(1)*inv_Ld;v_app(2)*inv_Lq]);

% Observer states
z1 = z1 + Ts*(f_nom + g_u + z2 - K1*sa1 - K2*sb1);
z2 = z2 + Ts*(-K3*sa2 - K4*sb2);
d_hat = z2;

% Precompute all eight dq voltage vectors

Vab = Kcl*V';
Vdq = single([ct, st; -st, ct])*Vab;

% Candidate-independent current prediction

id_base = is_d + TsLd*(-Rs*is_d + we*Lq*is_q) + Ts*d_hat(1);
iq_base = is_q + TsLq*(-Rs*is_q - we*Ld*is_d - we*lambda_f) + Ts*d_hat(2);

% Single-step FCS-MPC search

g_best = single(9e20);
idx    = int32(1);

id_best = single(0);
iq_best = single(0);

for n = 1:8

    % Predicted currents for switching candidate n
    id_p = id_base + TsLd*Vdq(1,n);
    iq_p = iq_base + TsLq*Vdq(2,n);

    % Current tracking errors
    ed = id_ref-id_p;
    eq = iq_ref-iq_p;

    % Cost function
    g = ed*ed + lambda_c*(eq*eq);

    if g < g_best
        g_best  = g;
        idx     = int32(n);
        id_best = id_p;
        iq_best = iq_p;
    end
end

% Selected switching state

s_prev = V(idx,:)';

Sa = s_prev(1);
Sb = s_prev(2);
Sc = s_prev(3);

gg = single([Sa;1-Sa;Sb;1-Sb;Sc;1-Sc]);
i_pred = single([id_best; iq_best]);

end

== matlab function Maxom_fcs_noncascaded/f_pmsm_foc_sl/MATLAB Function ==
  data: iq_ref output; we input; we_ref input; Te input; wm input; Kps input; Kis input; lambda_f input; Jm input; Bfric input; zeta input; wn input; iq_max input; Tcur input; iq_unsat output; e_we output; TL_est output
function [iq_ref, iq_unsat, e_we, TL_est] = est_iq_ref_check( ...
    we, we_ref, Te, wm, Kps, Kis,...
    lambda_f, Jm, Bfric, zeta, wn, iq_max, Tcur)
%#codegen
% *** Set this block: Update method = Discrete, Sample time = Tcur ***
% Now takes Te (electromagnetic torque) + wm (MECHANICAL speed, rad/s),
% and reconstructs the LOAD torque before feeding it forward.
np   = single(7);
we   = single(we);   we_ref = single(we_ref);
Te   = single(Te);   wm     = 7*single(we);
lambda_f = single(lambda_f); Jm = single(Jm); Bfric = single(Bfric);
zeta = single(zeta); wn = single(wn); iq_max = single(iq_max);
Ts   = single(Tcur); Kp_we = single(Kps/np); Ki_we=single(Kis/np);
Kt = single(1.5)*np*lambda_f;
if Kt < single(1e-6), Kt = single(1e-6); end     % guard lambda_f = 0
den    = np*Kt;
%Kp_we  = (single(2)*zeta*wn*Jm - Bfric)/den;
%Ki_we  = (Jm*wn*wn)/den;
inv_Kt = single(1)/Kt;
persistent Ispd wm_prev TL_f
if isempty(Ispd)
    Ispd = single(0);  wm_prev = wm;  TL_f = single(0);
end
% --- reconstruct load torque from Te (torque balance) ---
% wm arrives ELECTRICAL (from the wrapped-derivative chain) -> to mechanical
wm_mech  = wm / np;                              % elec rad/s -> mech rad/s
dwm      = (wm_mech - wm_prev)/Ts;               % mech speed derivative (noisy!)
dwm      = max(min(dwm, single(5e4)), single(-5e4));  % clip stray deriv spikes
wm_prev  = wm_mech;
TL_raw   = Te - Jm*dwm - Bfric*wm_mech;          % T_L = Te - J*a - B*w
% low-pass the estimate (fc ~ speed-loop bandwidth); alpha = Ts/(Ts+tau)
fc     = wn/(single(2)*single(pi));              % cutoff near the loop BW
tau    = single(1)/(single(2)*single(pi)*fc);
alpha  = Ts/(Ts + tau);
TL_f   = TL_f + alpha*(TL_raw - TL_f);
TL_est = TL_f;
% --- PI + load feed-forward ---
Kaw = Ki_we / Kp_we;
e_we     = we_ref - we;
iq_ff    = TL_est*inv_Kt;                        % now a LOAD term, not ~iq
iq_unsat = Kp_we*e_we + Ispd + iq_ff;
iq_ref   = max(min(iq_unsat, iq_max), -iq_max);
%% clamping anti-windup (no Kaw to blow up)
%hi = (iq_unsat >  iq_max) && (e_we > single(0));
%lo = (iq_unsat < -iq_max) && (e_we < single(0));
%if ~(hi || lo)
%    Ispd = Ispd + Ts*Ki_we*e_we;
%end
% back-calculation: keep integrating, bleed toward the achievable command
Ispd = Ispd + Ki_we*e_we + Ts*Kaw*(iq_ref - iq_unsat);
iq_ref = single(iq_ref); iq_unsat = single(iq_unsat);
e_we = single(e_we); TL_est = single(TL_est);
end

== matlab function Maxom_fcs_noncascaded/f_pmsm_foc_sl/MATLAB Function9 ==
  data: we input; we_dot output; Ts input
function we_dot = deriv(we, Ts)
%#codegen
persistent w_prev
if isempty(w_prev), w_prev = we; end
we_dot  = (we - w_prev) / Ts;
w_prev  = we;
end

== matlab function Maxom_fcs_noncascaded/f_pmsm_foc_sl/MATLAB Function1 ==
  data: speed_ref_cmd input; iq_feedforward output
function iq_feedforward = fcn_speed_feedforward( speed_ref_cmd)
    % ----------------- 系统硬参数定义 -----------------
    FS = single(32000);               % 控制频率 32kHz
    DT = single(1)/ FS;            % 采样周期 31.25us
    POLE_PAIRS = single(7);           % 极对数
    MAX_CURRENT_LIMIT = single(20); % 最大限流 20A (用于限制最大加速度)

    % ----------------- 电机软参数定义 (需要实测/辨识) -----------------
    % 1. J_total: 电机转子+负载的总转动惯量 (单位: kg·m^2)
    J_total = single(0.044e-4*2);        % 【需根据实际系统调整】
    % 2. Kt: 电机转矩常数 (单位: N·m/A)。通常 Kt ≈ 反电动势常数 Ke
    Kt = single(0.091003);                % 【需根据电机规格书调整】

    % ----------------- 持久化状态变量 -----------------
    persistent prev_ramped_speed ramped_speed
    if isempty(ramped_speed)
        prev_ramped_speed = single(0);
        ramped_speed = single(0);
    end

    persistent prev_iq_ff
if isempty(prev_iq_ff)
    prev_iq_ff = single(0);
end


    % ========================================================
    % 【第一步：速度轨迹规划（生成平滑斜坡）】
    % ========================================================
    % 理论最大加速度限制：a_max = (Kt * Max_Current) / J_total
    max_accel_rpm_s = (Kt * MAX_CURRENT_LIMIT) / J_total * 60.0 / (2 * pi);

    % 跟随目标速度（做斜坡上升/下降限制）
    if speed_ref_cmd > ramped_speed
        ramped_speed = ramped_speed + max_accel_rpm_s * DT; % 加速
        if ramped_speed > speed_ref_cmd
            ramped_speed = speed_ref_cmd;
        end
    elseif speed_ref_cmd < ramped_speed
        ramped_speed = ramped_speed - max_accel_rpm_s * DT; % 减速
        if ramped_speed < speed_ref_cmd
            ramped_speed = speed_ref_cmd;
        end
    end

    % ========================================================
    % 【第二步：计算加速度前馈】
    % ========================================================
    % 1. 计算速度差分（得到实际需要的加速度）
    delta_rpm = ramped_speed - prev_ramped_speed;
    accel_rpm_s = delta_rpm / DT; % RPM / s

    % 2. 将加速度转换为 电角速度 变化率 (rad/s^2)
    accel_rad_s2 = accel_rpm_s * (2 * pi / 60.0) * POLE_PAIRS;

    % 3. 计算所需的前馈 Iq 电流 (基于牛顿第二定律: T = J * a, T = Kt * Iq)
    iq_raw = (J_total * accel_rad_s2) / Kt;

    % --- 引入前馈斜率限制（替代低通滤波，0相位滞后） ---

% 设定前馈电流的最大变化率（单位：A/s）
% 根据电机电气时间常数，建议从 500 ~ 2000 A/s 开始往下调
MAX_FF_SLEW_RATE = single(50000); 
max_delta_per_loop = MAX_FF_SLEW_RATE * DT; % 每个控制周期允许的最大电流变化

diff = iq_raw - prev_iq_ff;
if diff > max_delta_per_loop
    diff = max_delta_per_loop;
elseif diff < -max_delta_per_loop
    diff = -max_delta_per_loop;
end

% 得到平滑后的前馈（方波的垂直边变成了斜坡边）
iq_feedforward = prev_iq_ff + diff;

% 最后统一做安全限幅
iq_feedforward = max(-MAX_CURRENT_LIMIT, min(MAX_CURRENT_LIMIT, iq_feedforward));
prev_iq_ff = iq_feedforward;

    % 4. 安全限幅（防止前馈计算出超出硬件能力的电流）
    if iq_feedforward > MAX_CURRENT_LIMIT
        iq_feedforward = MAX_CURRENT_LIMIT;
    elseif iq_feedforward < -MAX_CURRENT_LIMIT
        iq_feedforward = -MAX_CURRENT_LIMIT;
    end

    % 更新状态
    prev_ramped_speed = ramped_speed;
end

== matlab function Maxom_fcs_noncascaded/f_pmsm_foc_sl/MATLAB Function10 ==
  data: ia input; gg output; ib input; ic input; id_ref input; we_ref input; we input; TL_hat input; theta_m input; Vdc input; Ld input; Lq input; Rs input; lambda_f input; Jm input; Bfric input; Tcur input; lambda_id input; lambda_sw input; we_scale input; i_scale input; iq_max input; i_pred output; we_pred output; we_spread output
function [gg, i_pred, we_pred, we_spread] = fcs_noncascade_np3( ...
    ia, ib, ic, id_ref, we_ref, we, TL_hat, theta_m, ...
    Vdc, Ld, Lq, Rs, lambda_f, Jm, Bfric, Tcur, ...
    lambda_id, lambda_sw, we_scale, i_scale, iq_max)
%#codegen
% Non-cascade FCS-MPC, Np=3, full 8^3 enumeration, normalized cost.
% Optimized: constants hoisted, 8x8 switching table, speed update as MAC,
% per-step current recursion precomputed as affine (a*i + base).

np = single(7);
ia=single(ia); ib=single(ib); ic=single(ic);
id_ref=single(id_ref); we_ref=single(we_ref); we=single(we); TL_hat=single(TL_hat);
Vdc=single(Vdc); Ld=single(Ld); Lq=single(Lq); Rs=single(Rs); lambda_f=single(lambda_f);
Jm=single(Jm); Bfric=single(Bfric); Ts=single(Tcur);
lambda_id=single(lambda_id); lambda_sw=single(lambda_sw);
we_scale=single(we_scale); i_scale=single(i_scale); iq_max=single(iq_max);

theta_e = single(mod(np*theta_m - pi/2, 2*pi));
inv_Ld=single(1)/Ld; inv_Lq=single(1)/Lq; inv_J=single(1)/Jm;
TsLd=Ts*inv_Ld; TsLq=Ts*inv_Lq;
ct=single(cos(theta_e)); st=single(sin(theta_e));

% --- hoisted constants (were recomputed 512x) ---
Kt     = single(1.5)*np*lambda_f;     % torque constant
LdmLq  = Ld - Lq;                      % reluctance coeff
aRd    = single(1) - TsLd*Rs;          % id recursion: id_next = aRd*id + baseD + TsLd*Vdq
aRq    = single(1) - TsLq*Rs;          % iq recursion
TsKJ   = Ts*np*inv_J;                  % speed: we_next = aW*we + TsKJ*(Te - TL_hat)
aW     = single(1) - Ts*Bfric*inv_J;
inv_ws=single(1)/we_scale; inv_is=single(1)/i_scale;
imax2 = iq_max*iq_max; 
%imax2 = iq_max; 
BIGPEN=single(1e5);
lsw3  = lambda_sw/single(3);

% Clarke/Park (measured)
i_alpha=(single(2)/3)*(ia-single(0.5)*ib-single(0.5)*ic);
i_beta =(single(2)/3)*(single(sqrt(3))/2)*(ib-ic);
is_d= ct*i_alpha+st*i_beta;
is_q=-st*i_alpha+ct*i_beta;
x_k=single([is_d;is_q]);

% SMDO gains
AB=single(0.6); BB=single(1.2);
K1=single(6000); K2=single(6000); K3=single(2.5e5); K4=single(1e6);

V=single([0 0 0;1 0 0;1 1 0;0 1 0;0 1 1;0 0 1;1 0 1;1 1 1]);
Kcl=(single(2)/3)*Vdc*single([1 -0.5 -0.5;0 single(sqrt(3))/2 -single(sqrt(3))/2]);

persistent z1 z2 s_prev
if isempty(z1)
    z1=x_k; z2=zeros(2,1,'single'); s_prev=zeros(3,1,'single');
end

% ===== electrical SMDO update =====
th_p=theta_e-we*Ts; ctp=single(cos(th_p)); stp=single(sin(th_p));
v_app=single([ctp stp;-stp ctp])*(Kcl*s_prev);
e=z1-x_k; ae=abs(e); se=sign(e);
sa1=ae.^AB.*se; sb1=ae.^BB.*se;
sa2=ae.^(single(2)*AB-single(1)).*se; sb2=ae.^(single(2)*BB-single(1)).*se;
f_nom=single([(-Rs*x_k(1)+we*Lq*x_k(2))*inv_Ld; ...
              (-Rs*x_k(2)-we*Ld*x_k(1)-we*lambda_f)*inv_Lq]);
g_u=single([v_app(1)*inv_Ld; v_app(2)*inv_Lq]);
z1=z1+Ts*(f_nom+g_u+z2-K1*sa1-K2*sb1);
z2=z2+Ts*(-K3*sa2-K4*sb2);
bd = Ts*z2(1);   % constant per-step current bias (d)
bq = Ts*z2(2);   % (q)

% ===== 8 dq voltages, and per-vector current INCREMENTS =====
Vab=Kcl*V';
Vdq=single([ct st;-st ct])*Vab;      % 2x8
dVd = TsLd*Vdq(1,:);                  % 1x8 precomputed voltage->id increment
dVq = TsLq*Vdq(2,:);                  % 1x8

% ===== 8x8 switching table (leg changes n->m), + sw0 from s_prev =====
SW = zeros(8,8,'single');
for a=1:8
    for b=1:8
        SW(a,b)=abs(V(b,1)-V(a,1))+abs(V(b,2)-V(a,2))+abs(V(b,3)-V(a,3));
    end
end
sw0=zeros(8,1,'single');
for n=1:8
    sw0(n)=abs(V(n,1)-s_prev(1))+abs(V(n,2)-s_prev(2))+abs(V(n,3)-s_prev(3));
end

% ===== horizon-3 tree search =====
g_best=single(1e30); n1_best=int32(1);
id_best=single(0); iq_best=single(0); we_best1=single(0);
we_min1=single(1e30); we_max1=single(-1e30);

for n1=1:8
    id1 = aRd*is_d + bd + dVd(n1);
    iq1 = aRq*is_q + bq + dVq(n1);
    Te1 = Kt*iq1; % since Lq=Ld, id=0 we dropped the reluctance term +(Ld-Lq)*id*iq/lambda_f)
    we1 = aW*we + TsKJ*(Te1 - TL_hat);
    if we1<we_min1, we_min1=we1; end
    if we1>we_max1, we_max1=we1; end
    ew=(we_ref-we1)*inv_ws; 
    ei=(id_ref-id1)*inv_is;
    c1 = ew*ew + lambda_id*(ei*ei) + lsw3*sw0(n1);
    if (id1*id1+iq1*iq1)>imax2, c1=c1+BIGPEN; end

    for n2=1:8
        id2 = aRd*id1 + bd + dVd(n2);
        iq2 = aRq*iq1 + bq + dVq(n2);
        Te2 = Kt*iq2;
        we2 = aW*we1 + TsKJ*(Te2 - TL_hat);
        ew=(we_ref-we2)*inv_ws; ei=(id_ref-id2)*inv_is;
        c12 = c1 + ew*ew + lambda_id*(ei*ei) + lsw3*SW(n1,n2);
        if (id2*id2+iq2*iq2)>imax2, c12=c12+BIGPEN; end

        for n3=1:8
            id3 = aRd*id2 + bd + dVd(n3);
            iq3 = aRq*iq2 + bq + dVq(n3);
            Te3 = Kt*iq3;
            we3 = aW*we2 + TsKJ*(Te3 - TL_hat);
            ew=(we_ref-we3)*inv_ws; 
            ei=(id_ref-id3)*inv_is;
            Jc = c12 + ew*ew + lambda_id*(ei*ei) + lsw3*SW(n2,n3);
            if (id3*id3+iq3*iq3)>imax2, Jc=Jc+BIGPEN; end

            if Jc<g_best
                g_best=Jc; n1_best=int32(n1);
                id_best=id1; iq_best=iq1; we_best1=we1;
            end
        end
    end
end

s_prev=V(n1_best,:)';
Sa=s_prev(1); Sb=s_prev(2); Sc=s_prev(3);
gg=single([Sa;1-Sa;Sb;1-Sb;Sc;1-Sc]);
i_pred=single([id_best;iq_best]);
we_pred=single(we_best1);
we_spread=single(we_max1-we_min1);
end

== matlab function Maxom_fcs_noncascaded/f_pmsm_foc_sl/MATLAB Function11 ==
  data: Te input; TL output; J input; wm_hat input
function TL = T_load(Te, J, wm_hat)

TL = Te - J*wm_hat; %supposed to have  - B*wm but Bfric = 0, so ne sud'ba

end

== matlab function Maxom_fcs_noncascaded/MATLAB Function ==
  data: theta input; T_dist output; w input
function T_dist = fcn(theta, w)
    % 输入: theta(电机电角度/机械角度), w(电机转速 rad/s)
    % 输出: T_dist(叠加在Tm上的总扰动扭矩, 方向与运动相反)

    % --- 1. 参数定义 (建议放在外部结构体或持久变量中，此处仅为示例) ---
    % 库仑摩擦力矩 (常数)
    T_coulomb = single(0.05);   % N.m
    % 粘性摩擦系数
    B_viscous =single(0.0001);  % N.m/(rad/s)
    % 齿槽/纹波转矩幅值 (与位置相关)
    T_cogging_amp = single(0.2); % N.m
    % 电机极对数 (用于将机械角度转为电角度，若输入已是电角度则令 p=1)
    p = single(7); 

    % --- 2. 基于转速的扰动 (摩擦) ---
    % 使用 tanh 代替 sign 防止过零抖动 (数值稳定性更好)
    w_small = single(0.01); % 阈值
    if abs(w) < w_small
        % 静摩擦/爬行区线性化处理
        T_friction = (T_coulomb / w_small) * w; 
    else
        T_friction = T_coulomb * sign(w);
    end
    % 加粘性阻尼
    T_friction = T_friction + B_viscous * w;

    % --- 3. 基于位置的扰动 (齿槽转矩/负载周期性波动) ---
    % 例如：压缩机、活塞或偏心负载，扭矩随电角度周期变化
    theta_e = p * theta; % 电角度
    T_position_based = single(T_cogging_amp * sin(2 * theta_e)); % 2次谐波常见

    % --- 总扰动合成 (注意符号，通常抵抗运动) ---
    T_dist = T_friction + T_position_based; 
end
